simulink model "SMC_Observadores_chattering_VJJ"  (R2026b)
settings: Solver=ode4  StopTime=40  FixedStep=0.0001
settings Model: Creator=nestorhernandezcastellanos  LastModifiedBy=nestorhernandezcastellanos

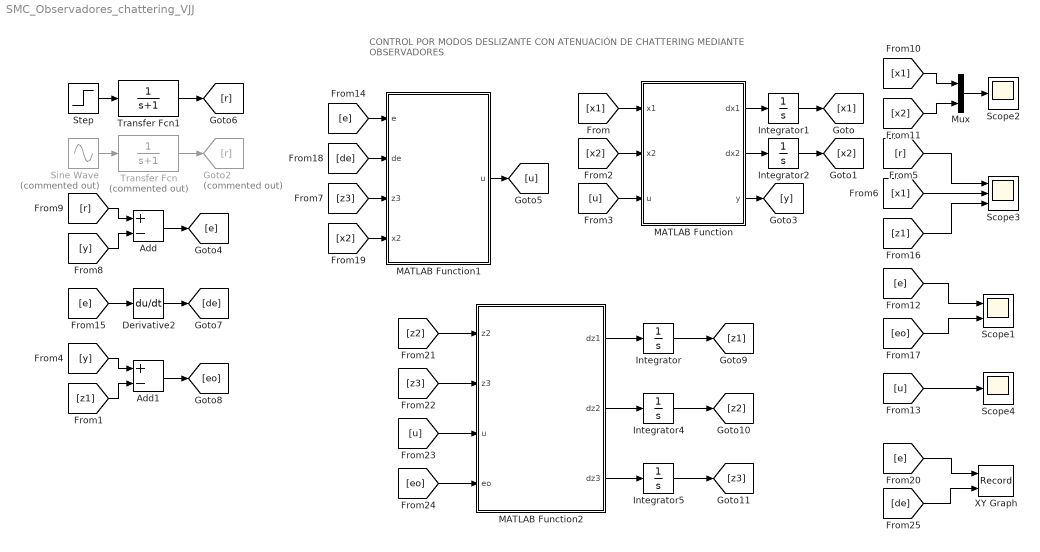
== system SMC_Observadores_chattering_VJJ ==
  note: CONTROL POR MODOS DESLIZANTE CON ATENUACIÓN DE CHATTERING MEDIANTE OBSERVADORES
  Add : Sum  Inputs=+-
  Add1 : Sum  Inputs=+-
  Derivative2 : Derivative
  Goto2 : Goto  Commented=on  GotoTag=r
  Integrator{,1..2,4..5} (5 alike) : Integrator
  MATLAB Function : MATLAB Function  TreatAsAtomicUnit=on
  MATLAB Function1 : MATLAB Function  TreatAsAtomicUnit=on
  MATLAB Function2 : MATLAB Function  TreatAsAtomicUnit=on
  Mux : Mux  Inputs=2
  Scope1 : Scope  NumInputPorts=2
      settings: ActiveDisplayYMinimum=-1.2750800139687928  ActiveDisplayYMaximum=1.2527866682187547
  Scope2 : Scope
      settings: ActiveDisplayYMinimum=-2.4390623918180623  ActiveDisplayYMaximum=1.9515615263625625  DataLoggingVariableName=ScopeData2
  Scope3 : Scope  NumInputPorts=3
      settings: ActiveDisplayYMinimum=-0.12585540371806453  ActiveDisplayYMaximum=1.1250950448569461  DataLoggingVariableName=ScopeData3
  Scope4 : Scope
      settings: ActiveDisplayYMinimum=-121.77408425670248  ActiveDisplayYMaximum=94.521077492843347
  Sine Wave : Sin  Commented=on  Amplitude=2  SampleTime=0
  Step : Step  Time=10  SampleTime=0
  Transfer Fcn : TransferFcn  Commented=on  Denominator=[1 1]
  Transfer Fcn1 : TransferFcn  Denominator=[1 1]
  XY Graph : Record  NumPorts=2.0  FileSettingsInternal="{\"entries\":[{\"content\":{\"excelSettings\":{\"content\":{},\"type\":\"Streamout.ExcelSettings\"},\"parquetSettings\":{\"content\":{},\"type\":\"Streamout.ParquetSettings\"}},\"type\":\"Streamout.FileSettingStorage\",\"uuid\":\"\"}],\"packageUris\":[\"http:\\/\\/schema.mathworks.com\\/mf0\\/streamout_blocks\\/R2020a\"],\"version\":\"1.0\"}"  FrameSettings=[0, 0]  Layout=[1 1]  SignalsInternal="{\"entries\":[{\"content\":{\"signals\":[{\"content\":{\"blockPath\":[],\"dimensions\":[1],\"domain\":\"\",\"lineColor\":\"#a2142f\",\"plots\":[ 1 ],\"port\":1,\"sid\":[\"\"],\"signalID\":1,\"signalName\":\"From20\"},\"type\":\"RecordBlkView.Signal\",\"uuid\":\"\"},{\"content\":{\"blockPath\":[],\"dimensions\":[1],\"domain\":\"\",\"lineColor\":\"#139fff\",\"plots\":[ 1 ],\"port\":2,\"sid\":[\"\"],\"signalID\":2,\"signalName\":\"From25\"},\"type\":\"RecordBlkView.Signal\",\"uuid\":\"\"}]},\"type\":\"RecordBlkView.InputSignals\",\"uuid\":\"\"}],\"packageUris\":[\"http:\\/\\/schema.mathworks.com\\/mf0\\/streamout_blocks\\/R2020a\"],\"version\":\"1.0\"}"  VisualizationBindings="{\"xyplotplugin\":{\"info\":[{\"series\":[{\"bindingParametersList\":[{\"parameter\":\"X-Axis\",\"signalID\":1,\"signalName\":\"From20\"},{\"parameter\":\"Y-Axis\",\"signalID\":2,\"signalName\":\"From25\"}],\"seriesID\":0}],\"subplotID\":1}]}}"  CompatibilityTag=XY
  wires:
  MATLAB Function/2(dx2) -> Integrator2/1
  MATLAB Function/1(dx1) -> Integrator1/1
  Mux/1 -> Scope2/1
  [de] -> MATLAB Function1/2(de)
  [x1] -> MATLAB Function/1(x1)
  [x2] -> MATLAB Function/2(x2)
  [r] -> Scope3/1
  [x1] -> Scope3/2
  Integrator2/1 -> [x2]
  Integrator1/1 -> [x1]
  MATLAB Function/3(y) -> [y]
  [y] -> Add/2
  [r] -> Add/1
  [x2] -> Mux/2
  [x1] -> Mux/1
  [e] -> Scope1/1
  [u] -> Scope4/1
  Add/1 -> [e]
  [e] -> MATLAB Function1/1(e)
  Step/1 -> Transfer Fcn1/1
  [e] -> Derivative2/1
  Derivative2/1 -> [de]
  MATLAB Function2/1(dz1) -> Integrator/1
  MATLAB Function2/2(dz2) -> Integrator4/1
  MATLAB Function2/3(dz3) -> Integrator5/1
  Integrator/1 -> [z1]
  Integrator4/1 -> [z2]
  Integrator5/1 -> [z3]
  [z2] -> MATLAB Function2/1(z2)
  [z3] -> MATLAB Function2/2(z3)
  [u] -> MATLAB Function2/3(u)
  [eo] -> MATLAB Function2/4(eo)
  Sine Wave/1 -> Transfer Fcn/1
  Transfer Fcn/1 -> Goto2/1
  MATLAB Function1/1(u) -> [u]
  [u] -> MATLAB Function/3(u)
  Transfer Fcn1/1 -> [r]
  Add1/1 -> [eo]
  [y] -> Add1/1
  [z1] -> Add1/2
  [z3] -> MATLAB Function1/3(z3)
  [z1] -> Scope3/3
  [eo] -> Scope1/2
  [x2] -> MATLAB Function1/4(x2)
  [e] -> XY Graph/1
  [de] -> XY Graph/2

== matlab function SMC_Observadores_chattering_VJJ/MATLAB Function1 ==
  data: e input; de input; z3 input; u output; x2 input
function u  = controlador(e, de, z3, x2)

m = 1;
K = 1;
b = 1;

% Superficie de deslizamiento
sigma = de + m*e;

% Ley de control
u = (-z3 - m*x2 + K*sign(sigma))/b;

== matlab function SMC_Observadores_chattering_VJJ/MATLAB Function ==
  data: x1 input; x2 input; dx1 output; u input; dx2 output; y output
function [dx1, dx2, y] = planta(x1, x2, u)

dx1 = x2;
dx2 = sin(x1*x2) + cos(x1+x2) + u;

y = x1;

== matlab function SMC_Observadores_chattering_VJJ/MATLAB Function2 ==
  data: z2 input; z3 input; u input; dz1 output; eo input; dz2 output; dz3 output
function [dz1, dz2, dz3] = LESO(z2, z3, u, eo)

b=1;

Ko1 = 45.9089;
Ko2 = 1156.247;
Ko3 = 8654.473;

% Observador
dz1 = z2 + Ko1*eo;
dz2 = z3 + b*u + Ko2*eo;
dz3 = Ko3*eo;
